simulink library "lib_LargeBuildingModel"  (R2026a)
settings: Solver=VariableStepAuto
libraries: WallSelector_lib x380, ExternalWall_lib x188, RoomWithAirVolume x140, fl_lib x139, RoomLevelControl_lib x1
(part 12 of 12)

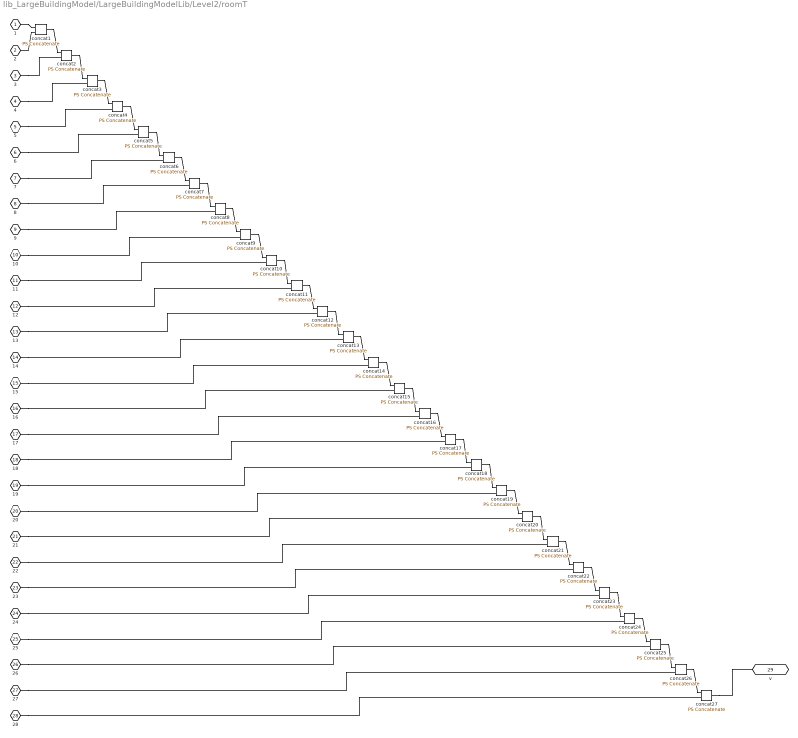
== system lib_LargeBuildingModel/LargeBuildingModelLib/Level2/roomT ==
  concat{1..27} (27 alike) : fl_lib/Physical Signals/Functions/PS Concatenate  catColumns=true
  1 : PMIOPort  Side=Left
  2 : PMIOPort  Port=2  Side=Left
  3 : PMIOPort  Port=3  Side=Left
  4 : PMIOPort  Port=4  Side=Left
  5 : PMIOPort  Port=5  Side=Left
  6 : PMIOPort  Port=6  Side=Left
  7 : PMIOPort  Port=7  Side=Left
  8 : PMIOPort  Port=8  Side=Left
  9 : PMIOPort  Port=9  Side=Left
  10 : PMIOPort  Port=10  Side=Left
  11 : PMIOPort  Port=11  Side=Left
  12 : PMIOPort  Port=12  Side=Left
  13 : PMIOPort  Port=13  Side=Left
  14 : PMIOPort  Port=14  Side=Left
  15 : PMIOPort  Port=15  Side=Left
  16 : PMIOPort  Port=16  Side=Left
  17 : PMIOPort  Port=17  Side=Left
  18 : PMIOPort  Port=18  Side=Left
  19 : PMIOPort  Port=19  Side=Left
  20 : PMIOPort  Port=20  Side=Left
  21 : PMIOPort  Port=21  Side=Left
  22 : PMIOPort  Port=22  Side=Left
  23 : PMIOPort  Port=23  Side=Left
  24 : PMIOPort  Port=24  Side=Left
  25 : PMIOPort  Port=25  Side=Left
  26 : PMIOPort  Port=26  Side=Left
  27 : PMIOPort  Port=27  Side=Left
  28 : PMIOPort  Port=28  Side=Left
  v : PMIOPort  Port=29  Side=Right
  connections:
  1/RConn1 -- concat1/LConn1
  2/RConn1 -- concat1/LConn2
  concat1/RConn1 -- concat2/LConn1
  3/RConn1 -- concat2/LConn2
  concat2/RConn1 -- concat3/LConn1
  4/RConn1 -- concat3/LConn2
  concat3/RConn1 -- concat4/LConn1
  5/RConn1 -- concat4/LConn2
  concat4/RConn1 -- concat5/LConn1
  6/RConn1 -- concat5/LConn2
  concat5/RConn1 -- concat6/LConn1
  7/RConn1 -- concat6/LConn2
  concat6/RConn1 -- concat7/LConn1
  8/RConn1 -- concat7/LConn2
  concat7/RConn1 -- concat8/LConn1
  9/RConn1 -- concat8/LConn2
  concat8/RConn1 -- concat9/LConn1
  10/RConn1 -- concat9/LConn2
  concat9/RConn1 -- concat10/LConn1
  11/RConn1 -- concat10/LConn2
  concat10/RConn1 -- concat11/LConn1
  12/RConn1 -- concat11/LConn2
  concat11/RConn1 -- concat12/LConn1
  13/RConn1 -- concat12/LConn2
  concat12/RConn1 -- concat13/LConn1
  14/RConn1 -- concat13/LConn2
  concat13/RConn1 -- concat14/LConn1
  15/RConn1 -- concat14/LConn2
  concat14/RConn1 -- concat15/LConn1
  16/RConn1 -- concat15/LConn2
  concat15/RConn1 -- concat16/LConn1
  17/RConn1 -- concat16/LConn2
  concat16/RConn1 -- concat17/LConn1
  18/RConn1 -- concat17/LConn2
  concat17/RConn1 -- concat18/LConn1
  19/RConn1 -- concat18/LConn2
  concat18/RConn1 -- concat19/LConn1
  20/RConn1 -- concat19/LConn2
  concat19/RConn1 -- concat20/LConn1
  21/RConn1 -- concat20/LConn2
  concat20/RConn1 -- concat21/LConn1
  22/RConn1 -- concat21/LConn2
  concat21/RConn1 -- concat22/LConn1
  23/RConn1 -- concat22/LConn2
  concat22/RConn1 -- concat23/LConn1
  24/RConn1 -- concat23/LConn2
  concat23/RConn1 -- concat24/LConn1
  25/RConn1 -- concat24/LConn2
  concat24/RConn1 -- concat25/LConn1
  26/RConn1 -- concat25/LConn2
  concat25/RConn1 -- concat26/LConn1
  27/RConn1 -- concat26/LConn2
  concat26/RConn1 -- concat27/LConn1
  28/RConn1 -- concat27/LConn2
  concat27/RConn1 -- v/RConn1

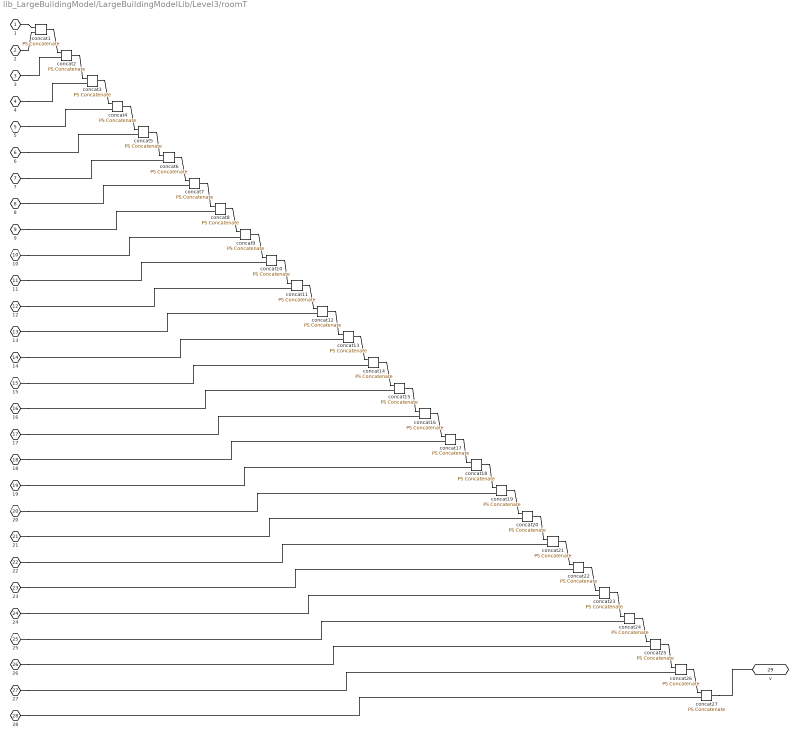
== system lib_LargeBuildingModel/LargeBuildingModelLib/Level3/roomT ==
  concat{1..27} (27 alike) : fl_lib/Physical Signals/Functions/PS Concatenate  catColumns=true
  1 : PMIOPort  Side=Left
  2 : PMIOPort  Port=2  Side=Left
  3 : PMIOPort  Port=3  Side=Left
  4 : PMIOPort  Port=4  Side=Left
  5 : PMIOPort  Port=5  Side=Left
  6 : PMIOPort  Port=6  Side=Left
  7 : PMIOPort  Port=7  Side=Left
  8 : PMIOPort  Port=8  Side=Left
  9 : PMIOPort  Port=9  Side=Left
  10 : PMIOPort  Port=10  Side=Left
  11 : PMIOPort  Port=11  Side=Left
  12 : PMIOPort  Port=12  Side=Left
  13 : PMIOPort  Port=13  Side=Left
  14 : PMIOPort  Port=14  Side=Left
  15 : PMIOPort  Port=15  Side=Left
  16 : PMIOPort  Port=16  Side=Left
  17 : PMIOPort  Port=17  Side=Left
  18 : PMIOPort  Port=18  Side=Left
  19 : PMIOPort  Port=19  Side=Left
  20 : PMIOPort  Port=20  Side=Left
  21 : PMIOPort  Port=21  Side=Left
  22 : PMIOPort  Port=22  Side=Left
  23 : PMIOPort  Port=23  Side=Left
  24 : PMIOPort  Port=24  Side=Left
  25 : PMIOPort  Port=25  Side=Left
  26 : PMIOPort  Port=26  Side=Left
  27 : PMIOPort  Port=27  Side=Left
  28 : PMIOPort  Port=28  Side=Left
  v : PMIOPort  Port=29  Side=Right
  connections:
  1/RConn1 -- concat1/LConn1
  2/RConn1 -- concat1/LConn2
  concat1/RConn1 -- concat2/LConn1
  3/RConn1 -- concat2/LConn2
  concat2/RConn1 -- concat3/LConn1
  4/RConn1 -- concat3/LConn2
  concat3/RConn1 -- concat4/LConn1
  5/RConn1 -- concat4/LConn2
  concat4/RConn1 -- concat5/LConn1
  6/RConn1 -- concat5/LConn2
  concat5/RConn1 -- concat6/LConn1
  7/RConn1 -- concat6/LConn2
  concat6/RConn1 -- concat7/LConn1
  8/RConn1 -- concat7/LConn2
  concat7/RConn1 -- concat8/LConn1
  9/RConn1 -- concat8/LConn2
  concat8/RConn1 -- concat9/LConn1
  10/RConn1 -- concat9/LConn2
  concat9/RConn1 -- concat10/LConn1
  11/RConn1 -- concat10/LConn2
  concat10/RConn1 -- concat11/LConn1
  12/RConn1 -- concat11/LConn2
  concat11/RConn1 -- concat12/LConn1
  13/RConn1 -- concat12/LConn2
  concat12/RConn1 -- concat13/LConn1
  14/RConn1 -- concat13/LConn2
  concat13/RConn1 -- concat14/LConn1
  15/RConn1 -- concat14/LConn2
  concat14/RConn1 -- concat15/LConn1
  16/RConn1 -- concat15/LConn2
  concat15/RConn1 -- concat16/LConn1
  17/RConn1 -- concat16/LConn2
  concat16/RConn1 -- concat17/LConn1
  18/RConn1 -- concat17/LConn2
  concat17/RConn1 -- concat18/LConn1
  19/RConn1 -- concat18/LConn2
  concat18/RConn1 -- concat19/LConn1
  20/RConn1 -- concat19/LConn2
  concat19/RConn1 -- concat20/LConn1
  21/RConn1 -- concat20/LConn2
  concat20/RConn1 -- concat21/LConn1
  22/RConn1 -- concat21/LConn2
  concat21/RConn1 -- concat22/LConn1
  23/RConn1 -- concat22/LConn2
  concat22/RConn1 -- concat23/LConn1
  24/RConn1 -- concat23/LConn2
  concat23/RConn1 -- concat24/LConn1
  25/RConn1 -- concat24/LConn2
  concat24/RConn1 -- concat25/LConn1
  26/RConn1 -- concat25/LConn2
  concat25/RConn1 -- concat26/LConn1
  27/RConn1 -- concat26/LConn2
  concat26/RConn1 -- concat27/LConn1
  28/RConn1 -- concat27/LConn2
  concat27/RConn1 -- v/RConn1

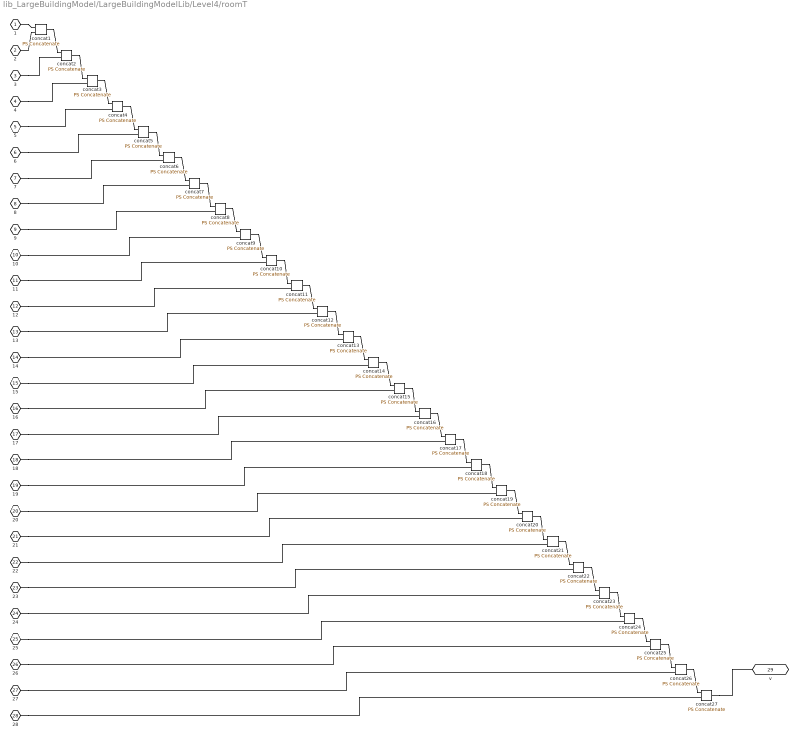
== system lib_LargeBuildingModel/LargeBuildingModelLib/Level4/roomT ==
  concat{1..27} (27 alike) : fl_lib/Physical Signals/Functions/PS Concatenate  catColumns=true
  1 : PMIOPort  Side=Left
  2 : PMIOPort  Port=2  Side=Left
  3 : PMIOPort  Port=3  Side=Left
  4 : PMIOPort  Port=4  Side=Left
  5 : PMIOPort  Port=5  Side=Left
  6 : PMIOPort  Port=6  Side=Left
  7 : PMIOPort  Port=7  Side=Left
  8 : PMIOPort  Port=8  Side=Left
  9 : PMIOPort  Port=9  Side=Left
  10 : PMIOPort  Port=10  Side=Left
  11 : PMIOPort  Port=11  Side=Left
  12 : PMIOPort  Port=12  Side=Left
  13 : PMIOPort  Port=13  Side=Left
  14 : PMIOPort  Port=14  Side=Left
  15 : PMIOPort  Port=15  Side=Left
  16 : PMIOPort  Port=16  Side=Left
  17 : PMIOPort  Port=17  Side=Left
  18 : PMIOPort  Port=18  Side=Left
  19 : PMIOPort  Port=19  Side=Left
  20 : PMIOPort  Port=20  Side=Left
  21 : PMIOPort  Port=21  Side=Left
  22 : PMIOPort  Port=22  Side=Left
  23 : PMIOPort  Port=23  Side=Left
  24 : PMIOPort  Port=24  Side=Left
  25 : PMIOPort  Port=25  Side=Left
  26 : PMIOPort  Port=26  Side=Left
  27 : PMIOPort  Port=27  Side=Left
  28 : PMIOPort  Port=28  Side=Left
  v : PMIOPort  Port=29  Side=Right
  connections:
  1/RConn1 -- concat1/LConn1
  2/RConn1 -- concat1/LConn2
  concat1/RConn1 -- concat2/LConn1
  3/RConn1 -- concat2/LConn2
  concat2/RConn1 -- concat3/LConn1
  4/RConn1 -- concat3/LConn2
  concat3/RConn1 -- concat4/LConn1
  5/RConn1 -- concat4/LConn2
  concat4/RConn1 -- concat5/LConn1
  6/RConn1 -- concat5/LConn2
  concat5/RConn1 -- concat6/LConn1
  7/RConn1 -- concat6/LConn2
  concat6/RConn1 -- concat7/LConn1
  8/RConn1 -- concat7/LConn2
  concat7/RConn1 -- concat8/LConn1
  9/RConn1 -- concat8/LConn2
  concat8/RConn1 -- concat9/LConn1
  10/RConn1 -- concat9/LConn2
  concat9/RConn1 -- concat10/LConn1
  11/RConn1 -- concat10/LConn2
  concat10/RConn1 -- concat11/LConn1
  12/RConn1 -- concat11/LConn2
  concat11/RConn1 -- concat12/LConn1
  13/RConn1 -- concat12/LConn2
  concat12/RConn1 -- concat13/LConn1
  14/RConn1 -- concat13/LConn2
  concat13/RConn1 -- concat14/LConn1
  15/RConn1 -- concat14/LConn2
  concat14/RConn1 -- concat15/LConn1
  16/RConn1 -- concat15/LConn2
  concat15/RConn1 -- concat16/LConn1
  17/RConn1 -- concat16/LConn2
  concat16/RConn1 -- concat17/LConn1
  18/RConn1 -- concat17/LConn2
  concat17/RConn1 -- concat18/LConn1
  19/RConn1 -- concat18/LConn2
  concat18/RConn1 -- concat19/LConn1
  20/RConn1 -- concat19/LConn2
  concat19/RConn1 -- concat20/LConn1
  21/RConn1 -- concat20/LConn2
  concat20/RConn1 -- concat21/LConn1
  22/RConn1 -- concat21/LConn2
  concat21/RConn1 -- concat22/LConn1
  23/RConn1 -- concat22/LConn2
  concat22/RConn1 -- concat23/LConn1
  24/RConn1 -- concat23/LConn2
  concat23/RConn1 -- concat24/LConn1
  25/RConn1 -- concat24/LConn2
  concat24/RConn1 -- concat25/LConn1
  26/RConn1 -- concat25/LConn2
  concat25/RConn1 -- concat26/LConn1
  27/RConn1 -- concat26/LConn2
  concat26/RConn1 -- concat27/LConn1
  28/RConn1 -- concat27/LConn2
  concat27/RConn1 -- v/RConn1
